simulink model "ob_buck"  (R2021a)
settings: Solver=VariableStepAuto  StartTime=0.0  StopTime=3  RelTol=1e-3
undefined symbols (not defined in the file): C, L, L1, L2, R
libraries: spsSeriesRLCBranchLib x6, spsVoltageMeasurementLib x4, spsCurrentMeasurementLib x2, spsDCVoltageSourceLib x2, spsDiodeLib x2, spsMosfetLib x2, pid_lib x2, eePwmGenerator x2, spspowerguiLib x1
settings Model: Creator=Julio  LastModifiedBy=Julio

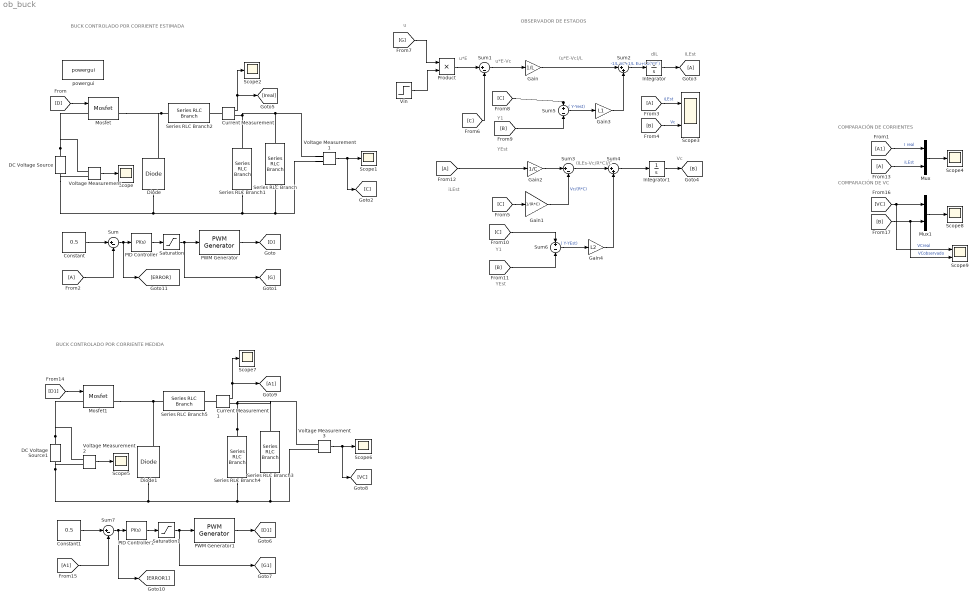
== system ob_buck ==
  note: (u*E-Vc)/L
  note: u
  note: Y1
  note: iLEst
  note: Vc
  note: YEst
  note: (iLEs-Vc/R*C)/C
  note: dIL
  note: iLEst
  note: YEst
  note: u*E
  note: Y1
  note: OBSERVADOR DE ESTADOS
  note: u*E-Vc
  note: COMPARACIÓN DE CORRIENTES
  note: BUCK CONTROLADO POR CORRIENTE ESTIMADA
  note: BUCK CONTROLADO POR CORRIENTE MEDIDA
  note: COMPARACIÓN DE VC
  Constant : Constant  Value=0.5
  Constant1 : Constant  Value=0.5
  Current Measurement : spsCurrentMeasurementLib/Current Measurement  PhasorSimulation=off  OutputType=Complex  PSBequivalent=0
  Current Measurement1 : spsCurrentMeasurementLib/Current Measurement  PhasorSimulation=off  OutputType=Complex  PSBequivalent=0
  DC Voltage Source : spsDCVoltageSourceLib/DC Voltage Source  Amplitude=24  Measurements=None
  DC Voltage Source1 : spsDCVoltageSourceLib/DC Voltage Source  Amplitude=24  Measurements=None
  Diode : spsDiodeLib/Diode  Ron=0.001  Lon=0  Vf=0.8  IC=0  UseSnubber=0  Rs=500  Cs=250e-9  Measurements=on
  Diode1 : spsDiodeLib/Diode  Ron=0.001  Lon=0  Vf=0.8  IC=0  UseSnubber=0  Rs=500  Cs=250e-9  Measurements=on
  Gain : Gain  Gain=1/L
  Gain1 : Gain  Gain=1/(R*C)
  Gain2 : Gain  Gain=1/C
  Gain3 : Gain  Gain=L1
  Gain4 : Gain  Gain=L2
  Integrator : Integrator
  Integrator1 : Integrator
  Mosfet : spsMosfetLib/Mosfet  Ron=0.1  Lon=0  Rd=0.01  Vfd=0  IC=0  Rs=1e5  Cs=inf  Measurements=on
  Mosfet1 : spsMosfetLib/Mosfet  Ron=0.1  Lon=0  Rd=0.01  Vfd=0  IC=0  Rs=1e5  Cs=inf  Measurements=on
  Mux : Mux  Inputs=2
  Mux1 : Mux  Inputs=2
  PID Controller : pid_lib/PID Controller  Controller=PI  Form=Parallel  TimeDomain=Continuous-time  UseExternalTs=off  SampleTime=-1  IntegratorMethod=Forward Euler  FilterMethod=Forward Euler  ControllerParametersSource=internal  P=200  I=0.1  D=0  UseFilter=on  N=100  TunerSelectOption=Transfer Function Based (PID Tuner App)  InitialConditionSource=internal  InitialConditionForIntegrator=0  InitialConditionForFilter=0  DifferentiatorICPrevScaledInput=0  ExternalReset=none  TrackingMode=off  Kt=1  LimitOutput=off  SatLimitsSource=internal  UpperSaturationLimit=inf  LowerSaturationLimit=-inf  LinearizeAsGain=on  AntiWindupMode=none  Kb=1  POutMin=[]  POutMax=[]  IOutMin=[]  IOutMax=[]  DOutMin=[]  DOutMax=[]  NOutMin=[]  NOutMax=[]  SumOutMin=[]  SumOutMax=[]  SaturationOutMin=[]  SaturationOutMax=[]  PParamMin=[]  PParamMax=[]  IParamMin=[]  IParamMax=[]  DParamMin=[]  DParamMax=[]  NParamMin=[]  NParamMax=[]  KbParamMin=[]  KbParamMax=[]  KtParamMin=[]  KtParamMax=[]  KbOutMin=[]  KbOutMax=[]  KtOutMin=[]  KtOutMax=[]  IntegratorOutMin=[]  IntegratorOutMax=[]  FilterOutMin=[]  FilterOutMax=[]  SumI1OutMin=[]  SumI1OutMax=[]  SumI2OutMin=[]  SumI2OutMax=[]  SumI3OutMin=[]  SumI3OutMax=[]  SumI4OutMin=[]  SumI4OutMax=[]  SumDOutMin=[]  SumDOutMax=[]  DifferentiatorOutMin=[]  DifferentiatorOutMax=[]  FilterDiffOutCoefMin=[]  FilterDiffOutCoefMax=[]  ReciprocalOutMin=[]  ReciprocalOutMax=[]  SumDenOutMin=[]  SumDenOutMax=[]  SumNumOutMin=[]  SumNumOutMax=[]  DivideOutMin=[]  DivideOutMax=[]  UdiffTsProdOutMin=[]  UdiffTsProdOutMax=[]  NTsProdOutMin=[]  NTsProdOutMax=[]  UintegralTsProdOutMin=[]  UintegralTsProdOutMax=[]  UngainTsProdOutMin=[]  UngainTsProdOutMax=[]  IntegratorContinuousStateAttributes=''  IntegratorStateMustResolveToSignalObject=off  IntegratorRTWStateStorageClass=Auto  FilterContinuousStateAttributes=''  FilterStateMustResolveToSignalObject=off  FilterRTWStateStorageClass=Auto  ParallelPVariant=InternalParameters  IdealPVariant=Disabled  IVariant=InternalParameters  DVariant=Disabled  IntegratorVariant=Continuous  SatVariant=Disabled  AWVariant=Passthrough  PCopyVariant=Disabled  TRVariant=Disabled  FdbkBlocksVariant=Forward  IdealPFdbkVariant=Disabled  SatFdbkVariant=Disabled  DerivativeFilterVariant=Disabled  NVariant=Disabled  NCopyVariant=Disabled_SignalSpec  FilterICVariant=Disabled  IntegratorICVariant=InternalICs  ExternalResetVariant=Disabled  TRSumVariant=Passthrough  SumFdbkVariant=Disabled  SumVariant=Sum_PI  TsampFilterVariant=InternalTs  TsampNgainVariant=Passthrough  TsampIntegralVariant=Passthrough  ExternalSaturationOutDataTypeStr=Inherit: Same as second input
  PID Controller1 : pid_lib/PID Controller  Controller=PI  Form=Parallel  TimeDomain=Continuous-time  UseExternalTs=off  SampleTime=-1  IntegratorMethod=Forward Euler  FilterMethod=Forward Euler  ControllerParametersSource=internal  P=200  I=0.1  D=0  UseFilter=on  N=100  TunerSelectOption=Transfer Function Based (PID Tuner App)  InitialConditionSource=internal  InitialConditionForIntegrator=0  InitialConditionForFilter=0  DifferentiatorICPrevScaledInput=0  ExternalReset=none  TrackingMode=off  Kt=1  LimitOutput=off  SatLimitsSource=internal  UpperSaturationLimit=inf  LowerSaturationLimit=-inf  LinearizeAsGain=on  AntiWindupMode=none  Kb=1  POutMin=[]  POutMax=[]  IOutMin=[]  IOutMax=[]  DOutMin=[]  DOutMax=[]  NOutMin=[]  NOutMax=[]  SumOutMin=[]  SumOutMax=[]  SaturationOutMin=[]  SaturationOutMax=[]  PParamMin=[]  PParamMax=[]  IParamMin=[]  IParamMax=[]  DParamMin=[]  DParamMax=[]  NParamMin=[]  NParamMax=[]  KbParamMin=[]  KbParamMax=[]  KtParamMin=[]  KtParamMax=[]  KbOutMin=[]  KbOutMax=[]  KtOutMin=[]  KtOutMax=[]  IntegratorOutMin=[]  IntegratorOutMax=[]  FilterOutMin=[]  FilterOutMax=[]  SumI1OutMin=[]  SumI1OutMax=[]  SumI2OutMin=[]  SumI2OutMax=[]  SumI3OutMin=[]  SumI3OutMax=[]  SumI4OutMin=[]  SumI4OutMax=[]  SumDOutMin=[]  SumDOutMax=[]  DifferentiatorOutMin=[]  DifferentiatorOutMax=[]  FilterDiffOutCoefMin=[]  FilterDiffOutCoefMax=[]  ReciprocalOutMin=[]  ReciprocalOutMax=[]  SumDenOutMin=[]  SumDenOutMax=[]  SumNumOutMin=[]  SumNumOutMax=[]  DivideOutMin=[]  DivideOutMax=[]  UdiffTsProdOutMin=[]  UdiffTsProdOutMax=[]  NTsProdOutMin=[]  NTsProdOutMax=[]  UintegralTsProdOutMin=[]  UintegralTsProdOutMax=[]  UngainTsProdOutMin=[]  UngainTsProdOutMax=[]  IntegratorContinuousStateAttributes=''  IntegratorStateMustResolveToSignalObject=off  IntegratorRTWStateStorageClass=Auto  FilterContinuousStateAttributes=''  FilterStateMustResolveToSignalObject=off  FilterRTWStateStorageClass=Auto  ParallelPVariant=InternalParameters  IdealPVariant=Disabled  IVariant=InternalParameters  DVariant=Disabled  IntegratorVariant=Continuous  SatVariant=Disabled  AWVariant=Passthrough  PCopyVariant=Disabled  TRVariant=Disabled  FdbkBlocksVariant=Forward  IdealPFdbkVariant=Disabled  SatFdbkVariant=Disabled  DerivativeFilterVariant=Disabled  NVariant=Disabled  NCopyVariant=Disabled_SignalSpec  FilterICVariant=Disabled  IntegratorICVariant=InternalICs  ExternalResetVariant=Disabled  TRSumVariant=Passthrough  SumFdbkVariant=Disabled  SumVariant=Sum_PI  TsampFilterVariant=InternalTs  TsampNgainVariant=Passthrough  TsampIntegralVariant=Passthrough  ExternalSaturationOutDataTypeStr=Inherit: Same as second input
  PWM Generator : eePwmGenerator/PWM Generator  CarrCount=Up  Tper=5e-5  Ts=5e-6
  PWM Generator1 : eePwmGenerator/PWM Generator  CarrCount=Up  Tper=5e-5  Ts=5e-6
  Product : Product
  Saturation : Saturate  UpperLimit=1  LowerLimit=0
  Saturation1 : Saturate  UpperLimit=1  LowerLimit=0
  Scope{,1..2,4..8} (8 alike) : Scope
  Scope3 : Scope  NumInputPorts=2
  Scope9 : Scope  NumInputPorts=2
  Series RLC Branch : spsSeriesRLCBranchLib/Series RLC Branch  LConnTagsString=__new0  RConnTagsString=__new0  BranchType=R  Resistance=10  Inductance=1e-3  SetiL0=off  InitialCurrent=0  Capacitance=1e-6  Setx0=off  InitialVoltage=0  Measurements=None
  Series RLC Branch1 : spsSeriesRLCBranchLib/Series RLC Branch  LConnTagsString=__new0  RConnTagsString=__new0  BranchType=C  Resistance=1  Inductance=1e-3  SetiL0=off  InitialCurrent=0  Capacitance=100e-6  Setx0=off  InitialVoltage=0  Measurements=None
  Series RLC Branch2 : spsSeriesRLCBranchLib/Series RLC Branch  LConnTagsString=__new0  RConnTagsString=__new0  BranchType=L  Resistance=1  Inductance=150e-3  SetiL0=off  InitialCurrent=0  Capacitance=1e-6  Setx0=off  InitialVoltage=0  Measurements=None
  Series RLC Branch3 : spsSeriesRLCBranchLib/Series RLC Branch  LConnTagsString=__new0  RConnTagsString=__new0  BranchType=R  Resistance=10  Inductance=1e-3  SetiL0=off  InitialCurrent=0  Capacitance=1e-6  Setx0=off  InitialVoltage=0  Measurements=None
  Series RLC Branch4 : spsSeriesRLCBranchLib/Series RLC Branch  LConnTagsString=__new0  RConnTagsString=__new0  BranchType=C  Resistance=1  Inductance=1e-3  SetiL0=off  InitialCurrent=0  Capacitance=100e-6  Setx0=off  InitialVoltage=0  Measurements=None
  Series RLC Branch5 : spsSeriesRLCBranchLib/Series RLC Branch  LConnTagsString=__new0  RConnTagsString=__new0  BranchType=L  Resistance=1  Inductance=150e-3  SetiL0=off  InitialCurrent=0  Capacitance=1e-6  Setx0=off  InitialVoltage=0  Measurements=None
  Sum{,1,3,7} (4 alike) : Sum  Inputs=|+-
  Sum2 : Sum  Inputs=|++
  Sum4 : Sum  Inputs=|++
  Sum5 : Sum  Inputs=+-
  Sum6 : Sum  Inputs=+-
  Vin : Step  After=24  SampleTime=0
  Voltage Measurement{,1..3} (4 alike) : spsVoltageMeasurementLib/Voltage Measurement  PhasorSimulation=off  OutputType=Complex  PSBequivalent=0
  powergui : spspowerguiLib/powergui  Priority=1  SimulationMode=Continuous  SampleTime=50e-6  frequency=60  Iterations=50  frequencyindice=0  Pbase=100e6  ErrMax=1e-4  UnitsV=kV  UnitsW=MW  buscounter=0  FunctionMessages=off  echomessages=off  EnableUseOfTLC=off  CurrentSourceSwitches=off  DisableSnubberDevices=off  DisableRonSwitches=off  DisableVfSwitches=off  DisplayEquations=off  AutomaticDiscreteSolvers=off  SolverType=Tustin/Backward Euler (TBE)  Interpol=off  ExternalGateDelay=off  methode=off  Ts=100  x0status=blocks  SPID=on  SwTol=0  HookPort=off  NonlinearTolerance=1e-4  nMaxIteration=100  ContinueOnMaxIteration=off  RestoreLinks=warning  ResistiveCurrentMeasurement=off  Frange=[0:2:500]  Ylog=off  Xlog=on  ShowGrid=off  save=off  variable=ZData  structure=0  ZoomFFT=off  StartTime=0.0  cycles=1  DisplayStyle=1  fundamental=60  FreqAxis=off  MaxFrequency=1000  frequencyindicesteady=1  RmsSteady=1  display=off
  wires:
  PWM Generator/1 -> [D]
  Sum/1 -> [ERROR], PID Controller/1
  Constant/1 -> Sum/1
  PID Controller/1 -> Saturation/1
  Voltage Measurement/1 -> Scope/1
  Voltage Measurement1/1 -> [C], Scope1/1
  Current Measurement/1 -> [Ireal], Scope2/1
  [C] -> Sum5/1
  [C] -> Gain1/1
  Vin/1 -> Product/2
  Sum3/1 -> Sum4/1
  Sum5/1 -> Gain3/1  "(\tY-Yest)"
  Integrator/1 -> [A]
  [B] -> Sum5/2
  Sum1/1 -> Gain/1
  [A] -> Scope3/1  "iLEst"
  [C] -> Sum1/2
  Sum4/1 -> Integrator1/1
  Gain3/1 -> Sum2/2
  Gain/1 -> Sum2/1
  [A] -> Gain2/1
  [B] -> Scope3/2  "Vc"
  [C] -> Sum6/1
  Gain1/1 -> Sum3/2  "Vc/(R*C)"
  Integrator1/1 -> [B]
  Sum6/1 -> Gain4/1  "(\tY-YEst)"
  Gain2/1 -> Sum3/1
  Gain4/1 -> Sum4/2
  [B] -> Sum6/2
  Sum2/1 -> Integrator/1  "-1/L Vc+1/L Eu+L1(Y-Y ̂)"
  Product/1 -> Sum1/1
  [G] -> Product/1
  [D] -> Mosfet/1
  [A] -> Sum/2
  Saturation/1 -> PWM Generator/1, [G]
  Mux/1 -> Scope4/1
  [A1] -> Mux/1  "I real"
  [A] -> Mux/2  "iLEst"
  [A1] -> Sum7/2
  [D1] -> Mosfet1/1
  PWM Generator1/1 -> [D1]
  Current Measurement1/1 -> [A1], Scope7/1
  Voltage Measurement2/1 -> Scope5/1
  Constant1/1 -> Sum7/1
  Voltage Measurement3/1 -> [VC], Scope6/1
  PID Controller1/1 -> Saturation1/1
  Sum7/1 -> [ERROR1], PID Controller1/1
  Saturation1/1 -> PWM Generator1/1, [G1]
  [VC] -> Scope9/1, Mux1/1  "VCreal"
  Mux1/1 -> Scope8/1
  [B] -> Scope9/2, Mux1/2  "VCobservado"
  connections:
  Series RLC Branch2/LConn1 -- Diode/RConn1 -- Mosfet/RConn1
  Series RLC Branch/LConn1 -- Voltage Measurement1/LConn1 -- Current Measurement/RConn1 -- Series RLC Branch1/LConn1
  DC Voltage Source/RConn1 -- Mosfet/LConn1 -- Voltage Measurement/LConn1
  Series RLC Branch1/RConn1 -- DC Voltage Source/LConn1 -- Voltage Measurement/LConn2 -- Diode/LConn1 -- Voltage Measurement1/LConn2 -- Series RLC Branch/RConn1
  Current Measurement/LConn1 -- Series RLC Branch2/RConn1
  DC Voltage Source1/RConn1 -- Mosfet1/LConn1 -- Voltage Measurement2/LConn1
  Series RLC Branch4/LConn1 -- Series RLC Branch3/LConn1 -- Voltage Measurement3/LConn1 -- Current Measurement1/RConn1
  Voltage Measurement2/LConn2 -- Series RLC Branch4/RConn1 -- Voltage Measurement3/LConn2 -- Series RLC Branch3/RConn1 -- Diode1/LConn1 -- DC Voltage Source1/LConn1
  Mosfet1/RConn1 -- Series RLC Branch5/LConn1 -- Diode1/RConn1
  Current Measurement1/LConn1 -- Series RLC Branch5/RConn1
